simulink model "L2"  (R2026b)
settings: Solver=VariableStepAuto
settings Model: Creator=v  LastModifiedBy=v

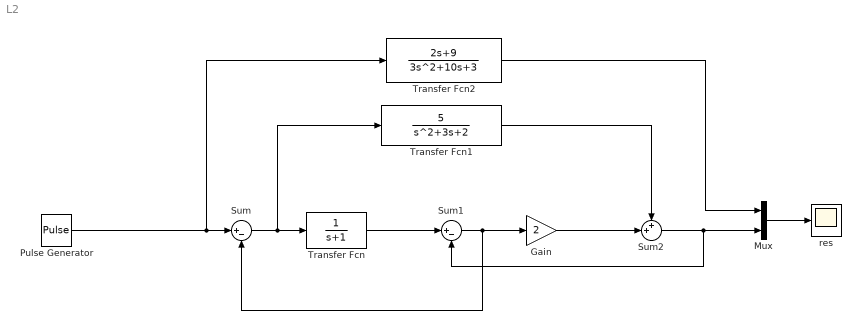
== system L2 ==
  Gain : Gain  Gain=2
  Mux : Mux  Inputs=2
  Pulse Generator : DiscretePulseGenerator  PulseType=Time based  Period=10  PulseWidth=5
  Sum : Sum  Inputs=|+-
  Sum1 : Sum  Inputs=|+-
  Sum2 : Sum  Inputs=++|
  Transfer Fcn : TransferFcn  Denominator=[1 1]
  Transfer Fcn1 : TransferFcn  Numerator=[5]  Denominator=[1 3 2]
  Transfer Fcn2 : TransferFcn  Numerator=[2 9]  Denominator=[3 10 3]
  res : Scope
      settings: ActiveDisplayYMinimum=-2.0670417771729159  ActiveDisplayYMaximum=5.3767784513022159
  wires:
  Pulse Generator/1 -> Sum/1, Transfer Fcn2/1
  Sum/1 -> Transfer Fcn1/1, Transfer Fcn/1
  Transfer Fcn/1 -> Sum1/1
  Gain/1 -> Sum2/2
  Transfer Fcn1/1 -> Sum2/1
  Sum2/1 -> Mux/2, Sum1/2
  Sum1/1 -> Sum/2, Gain/1
  Mux/1 -> res/1
  Transfer Fcn2/1 -> Mux/1
